simulink subsystem "Thrust_to_Mdot_LUT"  (R2026a)
settings: Solver=VariableStepAuto
undefined symbols (not defined in the file): fu_mdot_data, ox_mdot_data, thrust_data
settings Model: Creator=asing  LastModifiedBy=asing

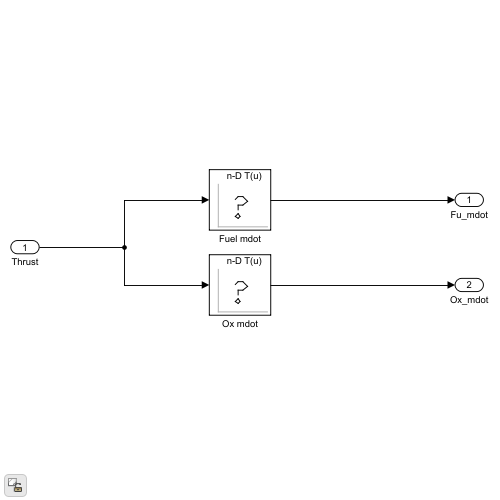
[thumbnail: Simulink's stored preview of the top-level diagram]
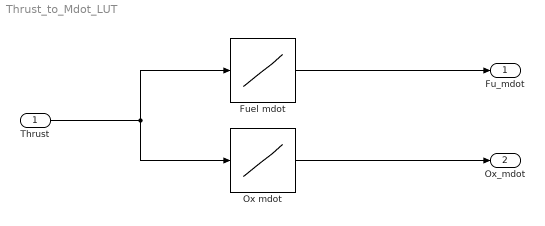
== system Thrust_to_Mdot_LUT ==
  Thrust : Inport
  Fuel mdot : Lookup_n-D  NumberOfTableDimensions=1  BreakpointsForDimension1=thrust_data  Table=fu_mdot_data  InternalRulePriority=Speed  RndMeth=Simplest
  Ox mdot : Lookup_n-D  NumberOfTableDimensions=1  BreakpointsForDimension1=thrust_data  Table=ox_mdot_data  InternalRulePriority=Speed  RndMeth=Simplest
  Fu_mdot : Outport
  Ox_mdot : Outport  Port=2
  wires:
  Thrust/1 -> Fuel mdot/1, Ox mdot/1
  Fuel mdot/1 -> Fu_mdot/1
  Ox mdot/1 -> Ox_mdot/1
